simulink model "test_SimulinkMdl2_qLPVMPCbeta_UIO_inside"  (R2020a)
settings: Solver=FixedStepAuto  StartTime=0.0  StopTime=400  FixedStep=DT  RelTol=1e-3
values from neighbouring files (symbols this model uses):
  betaLUT = 0.0 0.064193209888351435 0.11259119004615419 0.14929546421559495 0.18081611050661253 0.20926497731412011 0.23701571242082992 0.26197392072434883 0.28536133270107289 0.30770154712660031 0.32934362985133 0.35028758087526196 0.37035886727319672 0.38973202197033374 0.40858157789187255    [DD_test.sldd]    (also in exUIO_WECS.m = unique(Lin_points.Pitch))
  DT = 0.008    [LUTMFile.m]    (also in UIOLinestTr.m; exUIO_WECS.m; getFictInputMatricesOrd3M.m; initWorkspace.m)
  lambdaCqVecLUT = 0.0 6.127061506348616E-5 0.00012254123012697232 0.00018381184519045848 0.00024508246025394464 0.00030635307531743077 0.00036762369038091696 0.00042889430544440315 0.00049016492050788928 0.00055143553557137541 0.00061270615063486154 0.00067397676569834778 0.00073524738076183392 0.00079651799582532 0.00085778861088880629 0.00091905922595229242 0.00098032984101577856 0.0010416004560792648 0.001102871    [DD_test.sldd]    (also in exUIO_WECS.m = lambdaCqVecMin : dLlambdaCqVec:lambdaCqVecMax)
  lambdaTildaMat = 14.419529569316524 14.349603210880673 12.133085869773012 9.9 8.4 7.3000000000000007 6.5 5.8000000000000007 5.4 4.9 4.6000000000000005 4.3 4.1000000000000005 3.9000000000000004 3.7 13.719392614649337 13.574357234178933 11.313379017594022 9.2598290519250313 7.9268106449449158 6.9824653636911407 6.2259000594299776 5.6530125740384722 5.1921371802911152 4.81807621242771 4.4910785109643978 4.22716815598    [DD_test.sldd]    (also in exUIO_WECS.m = lambdaCqVecMax *ones(size(lambdaCqMat)))
  Lin_points = 0.74811652133345019 0.78122947334555715 0.82586806925039735 0.88042797952230989 0.94564154658981237 1.06231329175348 1.1780905557148451 1.2402773842094346 1.254474305465946 1.2544764615597244 1.2544775037226534 1.2544778841663968 1.2544780221694662 1.2544779823335293 1.254477987181289 1.2544781738200332 1.254478189259095 1.2544780953600987 1.2544781548505395 1.2544783366942183 1.2544785605869417 1    [DD_test.sldd]    (also in LinPointsMFile.m = struct)
  sysEstTr : value not decoded    [DD_test.sldd]
  sysMeasDel : value not decoded    [DD_test.sldd]
  wecs = 3.0    [DD_test.sldd]    (also in MdlMFile.m = struct)
undefined symbols (not defined in the file or in its folder): Rotor_Lambda
libraries: sharedTrackingLibrary x1
settings Model: DataDictionary=DD_test.sldd  ExtModeTrigMode=oneshot  ExtModeArmWhenConnect=off  Creator=Hazim Namik  LastModifiedBy=ditt_aj
settings DataIOCC: LimitDataPoints=on  SaveFormat=Array  ReturnWorkspaceOutputs=off
settings OptimizationCC: BlockReduction=off  BooleanDataType=off  LifeSpan=inf
settings DebuggingCC: SaveWithParameterizedLinksMsg=none  UnderspecifiedInitializationDetection=Classic  MergeDetectMultiDrivingBlocksExec=none  SignalResolutionControl=TryResolveAllWithWarning  SFUnexpectedBacktrackingDiag=warning  SFNoUnconditionalDefaultTransitionDiag=warning  SFExecutionAtInitializationDiag=none  ArithmeticOperatorsInVariantConditions=warning
settings HardwareCC: ProdBitPerPointer=32  ProdBitPerSizeT=32  ProdBitPerPtrDiffT=32  ProdLargestAtomicFloat=None  ProdIntDivRoundTo=Undefined  ProdEndianess=Unspecified  ProdWordSize=32  ProdHWDeviceType=32-bit Generic  TargetUnknown=on
settings ModelReferenceCC: PropagateSignalLabelsOutOfModel=off
settings SFSimCC: SimUseLocalCustomCode=off  CustomCodeUndefinedFunction=UseInterfaceOnly
settings RTWCC: RTWUseLocalCustomCode=off
settings CodeAppCC: StateflowObjectComments=on
settings GRTTargetCC: TargetLangStandard=C89/C90 (ANSI)
settings ConfigComp: CovMetricSettings=dw  CovHtmlReporting=on  CovSaveCumulativeToWorkspaceVar=on  CovSaveSingleToWorkspaceVar=on  CovExternalEMLEnable=off

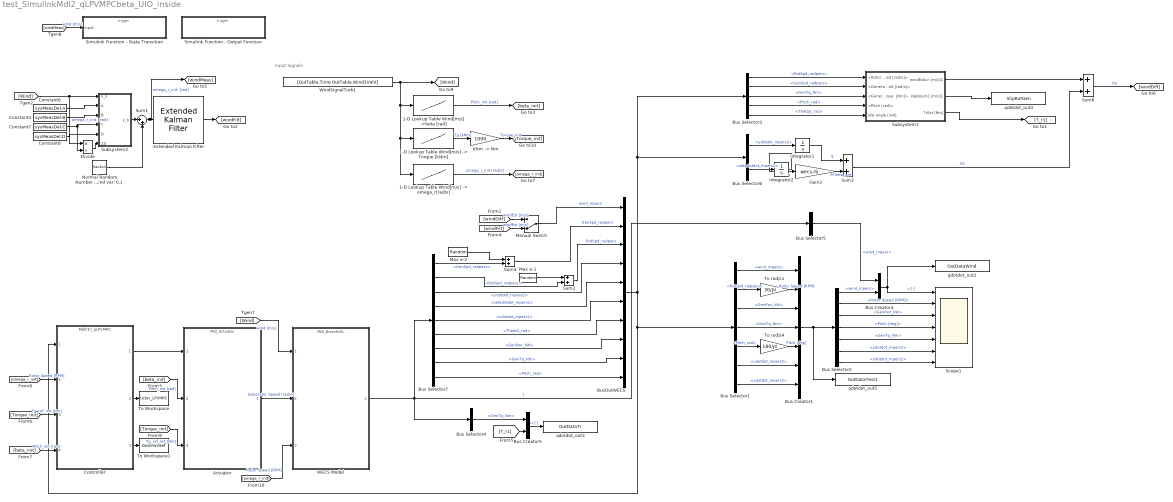
== system test_SimulinkMdl2_qLPVMPCbeta_UIO_inside ==
  note: Input Signals
  "1-D Lookup Table Wind[m/s] -> Torque [kNm]" : Lookup_n-D  NumberOfTableDimensions=1  BreakpointsForDimension1=Lin_points.V  BreakpointsForDimension2=Rotor_Lambda  Table=Lin_points.Torque  InternalRulePriority=Speed  RndMeth=Simplest  InputSameDT=on
  "1-D Lookup Table Wind[m/s] -> omega_r[rad/s]" : Lookup_n-D  NumberOfTableDimensions=1  BreakpointsForDimension1=Lin_points.V  BreakpointsForDimension2=Rotor_Lambda  Table=Lin_points.RSpeed  InternalRulePriority=Speed  RndMeth=Simplest  InputSameDT=on
  1-D Lookup Table Wind[m/s] ->beta [rad] : Lookup_n-D  NumberOfTableDimensions=1  BreakpointsForDimension1=Lin_points.V  BreakpointsForDimension2=Rotor_Lambda  Table=Lin_points.Pitch  InternalRulePriority=Speed  RndMeth=Simplest  InputSameDT=on
  Actuator : ModelReference  ModelNameDialog=Mdl_Actuator.slx  SimulationMode=Normal  ModelReferenceVersion=1.18
  Bus Creator1 : BusCreator  Inputs=7
  Bus Creator4 : BusCreator  Inputs=2
  Bus Creator5 : BusCreator  Inputs=2
  Bus Selector1 : BusSelector  OutputSignals=wind_mpers,RotSpd_radpers,GenPwr_kW,GenTq_Nm,Pitch_rad,ydotdot_mpers2,xdotdot_mpers2
  Bus Selector2 : BusSelector  OutputSignals=wind_mpers,Rotor Speed [RPM],GenPwr_kW,Pitch [deg],GenTq_Nm,ydotdot_mpers2,xdotdot_mpers2
  Bus Selector3 : BusSelector  OutputSignals=RotSpd_radpers,GenSpd_radpers,GenTq_Nm,Pitch_rad,ThetaS_rad
  Bus Selector4 : BusSelector  OutputSignals=GenTq_Nm
  Bus Selector5 : BusSelector  OutputSignals=wind_mpers
  Bus Selector6 : BusSelector  OutputSignals=ydotdot_mpers2,zetadotdot_mpers2
  Bus Selector7 : BusSelector  OutputSignals=GenSpd_radpers,RotSpd_radpers,ydotdot_mpers2,zetadotdot_mpers2,xdotdot_mpers2,ThetaS_rad,GenPwr_kW,GenTq_Nm,Pitch_rad
  BusOutWECS : BusCreator  Inputs=10  OutDataTypeStr=Bus: slBus1
  Constant4 : Constant  Value=sysMeasDel.B
  Constant6 : Constant  Value=sysMeasDel.A
  Constant7 : Constant  Value=sysMeasDel.C
  Constant8 : Constant  Value=sysMeasDel.D
  Controller : ModelReference  ModelNameDialog=MdlCtrl_qLPVMPC.slx  SimulationMode=Normal  ModelReferenceVersion=1.29
  Divide : Product  Inputs=*/
  Extended Kalman Filter : sharedTrackingLibrary/Extended Kalman Filter  StateTransitionFcn=stateTransitionFcn  HasStateTransitionJacobianFcn=off  StateTransitionJacobianFcn=stateTransitionJacobianFcn  HasAdditiveProcessNoise=Additive  ProcessNoise=0.1  HasTimeVaryingProcessNoise=off  HasStateTransitionFcnExtraArgument=0  InitialState=18  InitialStateCovariance=0.1  MeasurementFcn1=outputFcn  HasMeasurementJacobianFcn1=off  HasMeasurementEnablePort1=off  HasAdditiveMeasurementNoise1=Additive  MeasurementNoise1=1  HasTimeVaryingMeasurementNoise1=off  HasMeasurementFcnExtraArgument1=0  MeasurementFcn2=gpsMeasurementFcn  HasMeasurementJacobianFcn2=off  HasMeasurementEnablePort2=off  HasAdditiveMeasurementNoise2=Additive  MeasurementNoise2=[100 0; 0 100]  HasTimeVaryingMeasurementNoise2=off  HasMeasurementFcnExtraArgument2=0  MeasurementFcn3=myMeasurementFcn  HasMeasurementJacobianFcn3=off  HasMeasurementEnablePort3=off  HasAdditiveMeasurementNoise3=Additive  MeasurementNoise3=1  HasTimeVaryingMeasurementNoise3=off  HasMeasurementFcnExtraArgument3=0  MeasurementFcn4=myMeasurementFcn  HasMeasurementJacobianFcn4=off  HasMeasurementEnablePort4=off  HasAdditiveMeasurementNoise4=Additive  MeasurementNoise4=1  HasTimeVaryingMeasurementNoise4=off  HasMeasurementFcnExtraArgument4=0  MeasurementFcn5=myMeasurementFcn  HasMeasurementJacobianFcn5=off  HasMeasurementEnablePort5=off  HasAdditiveMeasurementNoise5=Additive  MeasurementNoise5=1  HasTimeVaryingMeasurementNoise5=off  HasMeasurementFcnExtraArgument5=0  EnableMultirate=off  StateTransitionFcnSampleTime=DT  MeasurementFcn1SampleTime=DT  MeasurementFcn2SampleTime=1  MeasurementFcn3SampleTime=-1  MeasurementFcn4SampleTime=-1  MeasurementFcn5SampleTime=-1  UseCurrentEstimator=off  OutputStateCovariance=off  DataType=double  SampleTime=DT  NumberOfMeasurements=1
      settings: SourceProductBaseCode=CT,DR,TF,ID,NV,AR,RO,VE
  Gain2 : Gain  Gain=wecs.rb
  Integrator1 : Integrator
  Integrator2 : Integrator
  Manual Switch : ManualSwitch  CurrentSetting=0
  Max e-1 : UniformRandomNumber  Minimum=-10^-4  Maximum=10^-4
  Max e-2 : UniformRandomNumber  Minimum=-10^-6  Maximum=10^-6
  Normal Random Number Wind var: 0.1 : RandomNumber  Variance=0.1  SampleTime=DT
  Scope1 : Scope  NumInputPorts=7
      settings: Tag=Scope
  Simulink Function - Output Function : Subsystem  TreatAsAtomicUnit=on
  Simulink Function - State Transition : Subsystem  TreatAsAtomicUnit=on
  Subsystem1 : Subsystem
  Subsystem2 : Subsystem
  Sum1 : Sum  Inputs=|++
  Sum{2..4,6} (4 alike) : Sum
  To Workspace : ToWorkspace  VariableName=tictoc_LPVMPC  SaveFormat=Timeseries  SampleTime=-1
  To Workspace1 : ToWorkspace  VariableName=GenPwrRef  SaveFormat=Timeseries  SampleTime=-1
  To rad/s1 : Gain  Gain=30/pi
  To rad/s4 : Gain  Gain=180/pi
  WECS Model : ModelReference  ModelNameDialog=Mdl_BianchiOL.slx  SimulationMode=Normal  ModelReferenceVersion=1.63
  WindSignalTurb1 : FromWorkspace  VariableName=[OutTable.Time OutTable.Wind1VelX]  SampleTime=DT  OutputAfterFinalValue=Holding final value
  "kNm -> Nm" : Gain  Gain=1000
  qdotdot_out2 : ToWorkspace  VariableName=OutDataWind  SampleTime=-1
  qdotdot_out3 : ToWorkspace  VariableName=OutDataTr  SampleTime=-1
  qdotdot_out4 : ToWorkspace  VariableName=SlipRotGen  SampleTime=-1
  qdotdot_out5 : ToWorkspace  VariableName=OutDataTest1  SampleTime=-1
  wires:
  WindSignalTurb1/1 -> [Wind], "1-D Lookup Table Wind[m/s] -> omega_r[rad/s]"/1, "1-D Lookup Table Wind[m/s] -> Torque [kNm]"/1, 1-D Lookup Table Wind[m/s] ->beta [rad]/1
  "kNm -> Nm"/1 -> [Torque_init]  "Torque_init"
  [omega_r_init] -> WECS Model/3  "Rotor Speed [RPM]"
  "1-D Lookup Table Wind[m/s] -> omega_r[rad/s]"/1 -> [omega_r_init]  "omega_r_init [rad/s]"
  [Wind] -> WECS Model/1  "wind [m/s]"
  1-D Lookup Table Wind[m/s] ->beta [rad]/1 -> [beta_init]  "Pitch_init [rad]"
  "1-D Lookup Table Wind[m/s] -> Torque [kNm]"/1 -> "kNm -> Nm"/1  "Tg [kNm]"
  Actuator/1 -> WECS Model/2  "Generator Speed [rad/s]"
  Controller/3 -> To Workspace1/1
  Bus Selector3/3 -> Subsystem1/3(<Generator Torque  [Nm]>)  "<GenTq_Nm>"
  Bus Selector3/4 -> Subsystem1/4(<Pitch [rad]>)  "<Pitch_rad>"
  Manual Switch/1 -> BusOutWECS/1  "wind_mpers"
  Bus Creator4/1 -> Scope1/1, qdotdot_out2/1  "u [-]"
  [Wind] -> Divide/1, Subsystem2/1(u_k)  "omega_r_init  [rad]"
  [windDiff] -> Manual Switch/1  "windEst [m/s]"
  Constant6/1 -> Subsystem2/2(A)
  Constant4/1 -> Subsystem2/3(B)
  Constant7/1 -> Subsystem2/4(C), Divide/2
  Constant8/1 -> Subsystem2/5(D)
  Divide/1 -> Subsystem2/6(Z0)
  Extended Kalman Filter/1 -> [windFilt]
  [windMeas] -> Simulink Function - State Transition/1(Input)  "wind [m/s]"
  Subsystem2/1(y_k) -> Sum1/1
  Sum1/1 -> [windMeas], Extended Kalman Filter/1  "omega_r_init  [rad]"
  Bus Selector3/5 -> Subsystem1/5(slip angle [rad])  "<ThetaS_rad>"
  Gain2/1 -> Sum3/2  "R*zeta_dot"
  Bus Selector6/1 -> Integrator1/1  "<ydotdot_mpers2>"
  Integrator1/1 -> Sum3/1  "q"
  Bus Selector6/2 -> Integrator2/1  "<zetadotdot_mpers2>"
  Integrator2/1 -> Gain2/1  "q"
  Sum3/1 -> Sum6/2  "Ve"
  Sum6/1 -> [windDiff]  "Ve"
  Subsystem1/1(windEstLin [m/s]1) -> Sum6/1
  Subsystem1/2(statesLIn2 [m/s]1) -> qdotdot_out4/1
  Subsystem1/3(TrEst [Nm]) -> [T_r1]
  Bus Creator5/1 -> qdotdot_out3/1  "u [-]"
  [T_r1] -> Bus Creator5/2
  Bus Selector3/2 -> Subsystem1/2(<Generator Speed [rad/s]>)  "<GenSpd_radpers>"
  Bus Selector3/1 -> Subsystem1/1(<Rotor Speed [rad/s]>)  "<RotSpd_radpers>"
  WECS Model/1 -> Bus Selector5/1, Bus Selector7/1, Bus Selector4/1  "]"
  [windFilt] -> Manual Switch/2  "windEst [m/s]"
  Normal Random Number Wind var: 0.1/1 -> Sum1/2
  Controller/2 -> To Workspace/1
  Controller/1 -> Actuator/1
  [beta_init] -> Actuator/2  "Pitch_init [rad]"
  [Torque_init] -> Actuator/3  "Tg_ref_init [Nm]"
  Bus Selector2/3 -> Scope1/3  "<GenPwr_kW>"
  Bus Selector2/7 -> Scope1/7  "<xdotdot_mpers2>"
  To rad/s4/1 -> Bus Creator1/5  "Pitch [deg]"
  Bus Selector2/4 -> Scope1/4  "<Pitch [deg]>"
  Bus Selector2/1 -> Bus Creator4/2  "<wind_mpers>"
  Bus Selector2/6 -> Scope1/6  "<ydotdot_mpers2>"
  Bus Selector1/5 -> To rad/s4/1  "<Pitch_rad>"
  Bus Selector1/4 -> Bus Creator1/4  "<GenTq_Nm>"
  Bus Selector2/2 -> Scope1/2  "<Rotor Speed [RPM]>"
  To rad/s1/1 -> Bus Creator1/2  "Rotor Speed [RPM]"
  Bus Selector1/6 -> Bus Creator1/6  "<ydotdot_mpers2>"
  Bus Selector2/5 -> Scope1/5  "<GenTq_Nm>"
  Bus Selector1/7 -> Bus Creator1/7  "<xdotdot_mpers2>"
  Bus Selector1/3 -> Bus Creator1/3  "<GenPwr_kW>"
  Max e-1/1 -> Sum2/1
  Bus Creator1/1 -> Bus Selector2/1, qdotdot_out5/1
  Max e-2/1 -> Sum4/1
  Bus Selector1/2 -> To rad/s1/1  "<RotSpd_radpers>"
  Bus Selector7/2 -> Sum2/2  "<RotSpd_radpers>"
  Bus Selector1/1 -> Bus Creator1/1  "<wind_mpers>"
  [Torque_init] -> Controller/3  "Tg_ref_init [Nm]"
  [beta_init] -> Controller/4  "Pitch_init [rad]"
  [omega_r_init] -> Controller/2  "Rotor Speed [RPM]"
  Bus Selector7/1 -> Sum4/2  "<GenSpd_radpers>"
  Sum4/1 -> BusOutWECS/2  "GenSpd_radpers"
  Sum2/1 -> BusOutWECS/3  "RotSpd_radpers"
  Bus Selector7/9 -> BusOutWECS/10  "<Pitch_rad>"
  Bus Selector7/8 -> BusOutWECS/9  "<GenTq_Nm>"
  Bus Selector7/7 -> BusOutWECS/8  "<GenPwr_kW>"
  Bus Selector7/6 -> BusOutWECS/7  "<ThetaS_rad>"
  Bus Selector7/5 -> BusOutWECS/6  "<xdotdot_mpers2>"
  Bus Selector7/4 -> BusOutWECS/5  "<zetadotdot_mpers2>"
  Bus Selector7/3 -> BusOutWECS/4  "<ydotdot_mpers2>"
  Bus Selector4/1 -> Bus Creator5/1  "<GenTq_Nm>"
  BusOutWECS/1 -> Bus Selector6/1, Bus Selector3/1, Bus Selector1/1, Controller/1
  Bus Selector5/1 -> Bus Creator4/1  "<wind_mpers>"

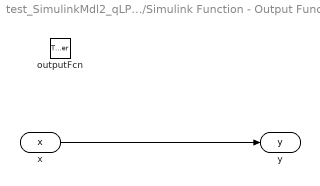
== system test_SimulinkMdl2_qLPVMPCbeta_UIO_inside/Simulink Function - Output Function ==
  outputFcn : TriggerPort  TriggerType=function-call  IsSimulinkFunction=on  FunctionName=outputFcn  VariantControl=Variant
  x : ArgIn  DisableCoverage=on  ArgumentName=x
  y : ArgOut  DisableCoverage=on  ArgumentName=y
  wires:
  x/1 -> y/1

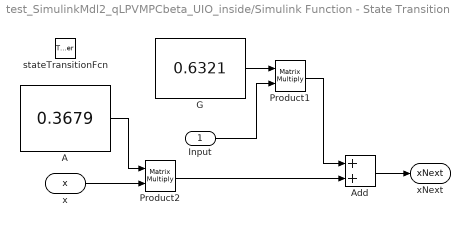
== system test_SimulinkMdl2_qLPVMPCbeta_UIO_inside/Simulink Function - State Transition ==
  Input : Inport
  stateTransitionFcn : TriggerPort  TriggerType=function-call  IsSimulinkFunction=on  FunctionName=stateTransitionFcn  VariantControl=Variant
  A : Constant  Value=0.3679
  Add : Sum
  G : Constant  Value=0.6321
  Product1 : Product  Multiplication=Matrix(*)
  Product2 : Product  Multiplication=Matrix(*)
  x : ArgIn  DisableCoverage=on  ArgumentName=x
  xNext : ArgOut  DisableCoverage=on  ArgumentName=xNext
  wires:
  x/1 -> Product2/2
  A/1 -> Product2/1
  Product2/1 -> Add/2
  G/1 -> Product1/1
  Input/1 -> Product1/2
  Product1/1 -> Add/1
  Add/1 -> xNext/1

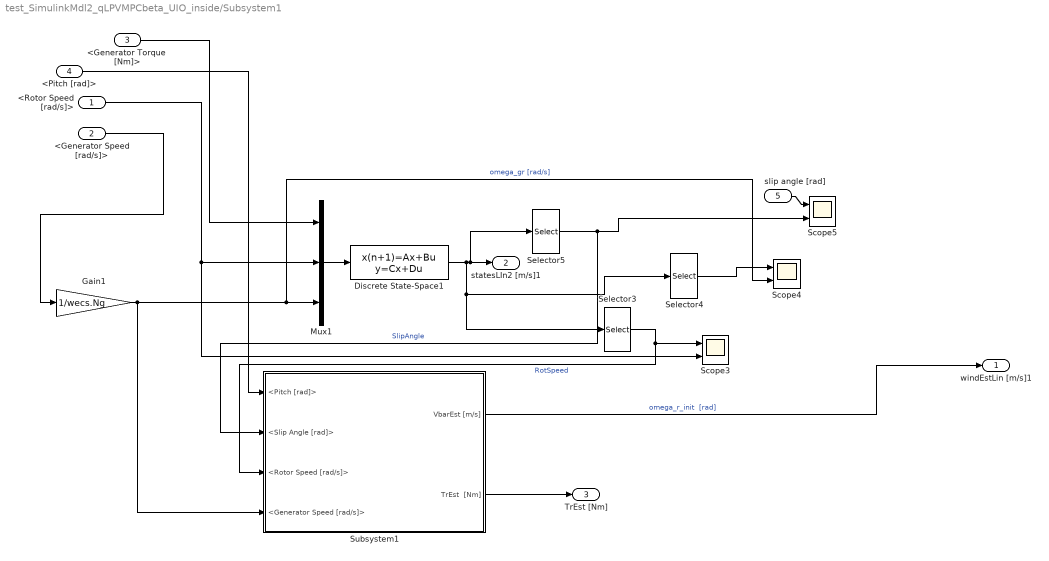
== system test_SimulinkMdl2_qLPVMPCbeta_UIO_inside/Subsystem1 ==
  <Rotor Speed [rad/s]> : Inport
  <Generator Speed [rad/s]> : Inport  Port=2
  <Generator Torque  [Nm]> : Inport  Port=3
  <Pitch [rad]> : Inport  Port=4
  slip angle [rad] : Inport  Port=5
  Discrete State-Space1 : DiscreteStateSpace  A=sysEstTr.A  B=sysEstTr.B  C=sysEstTr.C  D=sysEstTr.D  InitialCondition=[0,0,1.25]  SampleTime=DT
  Gain1 : Gain  Gain=1/wecs.Ng
  Mux1 : Mux  Inputs=3
  Scope3 : Scope  NumInputPorts=2
  Scope4 : Scope  NumInputPorts=2
  Scope5 : Scope  NumInputPorts=2
  Selector3 : Selector  InputPortWidth=3  IndexOptions=Index vector (dialog)  Indices=2  OutputSizes=1
  Selector4 : Selector  InputPortWidth=3  IndexOptions=Index vector (dialog)  Indices=3  OutputSizes=1
  Selector5 : Selector  InputPortWidth=3  IndexOptions=Index vector (dialog)  Indices=1  OutputSizes=1
  Subsystem1 : Subsystem
  windEstLin [m/s]1 : Outport
  statesLIn2 [m/s]1 : Outport  Port=2
  TrEst [Nm] : Outport  Port=3
  wires:
  <Generator Speed [rad/s]>/1 -> Gain1/1
  <Generator Torque  [Nm]>/1 -> Mux1/1
  <Pitch [rad]>/1 -> Subsystem1/1(<Pitch [rad]>)
  slip angle [rad]/1 -> Scope5/1
  Subsystem1/1(VbarEst [m/s]) -> windEstLin [m/s]1/1  "omega_r_init  [rad]"
  <Rotor Speed [rad/s]>/1 -> Mux1/2, Scope3/2
  Mux1/1 -> Discrete State-Space1/1
  Selector3/1 -> Subsystem1/3(<Rotor Speed [rad/s]>), Scope3/1  "RotSpeed"
  Gain1/1 -> Subsystem1/4(<Generator Speed [rad/s]>), Scope4/2, Mux1/3  "omega_gr [rad/s]"
  Discrete State-Space1/1 -> Selector5/1, statesLIn2 [m/s]1/1, Selector4/1, Selector3/1
  Selector4/1 -> Scope4/1
  Selector5/1 -> Subsystem1/2(<Slip Angle [rad]>), Scope5/2  "SlipAngle"
  Subsystem1/2(TrEst  [Nm]) -> TrEst [Nm]/1

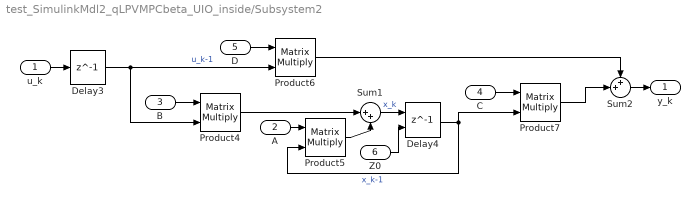
== system test_SimulinkMdl2_qLPVMPCbeta_UIO_inside/Subsystem2 ==
  u_k : Inport
  A : Inport  Port=2
  B : Inport  Port=3
  C : Inport  Port=4
  D : Inport  Port=5
  Z0 : Inport  Port=6
  Delay3 : Delay  DelayLength=1
  Delay4 : Delay  DelayLength=1  InitialConditionSource=Input port
      settings: InputPortMap=u0,p4
  Product{4..7} (4 alike) : Product  Multiplication=Matrix(*)
  Sum1 : Sum  Inputs=|++
  Sum2 : Sum  Inputs=++|
  y_k : Outport
  wires:
  Delay4/1 -> Product7/2, Product5/2  "x_k-1"
  u_k/1 -> Delay3/1
  Product7/1 -> Sum2/2
  C/1 -> Product7/1
  Product6/1 -> Sum2/1
  Delay3/1 -> Product4/2, Product6/2  "u_k-1"
  Product5/1 -> Sum1/2
  D/1 -> Product6/1
  Product4/1 -> Sum1/1
  A/1 -> Product5/1
  Sum1/1 -> Delay4/1  "x_k"
  B/1 -> Product4/1
  Sum2/1 -> y_k/1
  Z0/1 -> Delay4/2

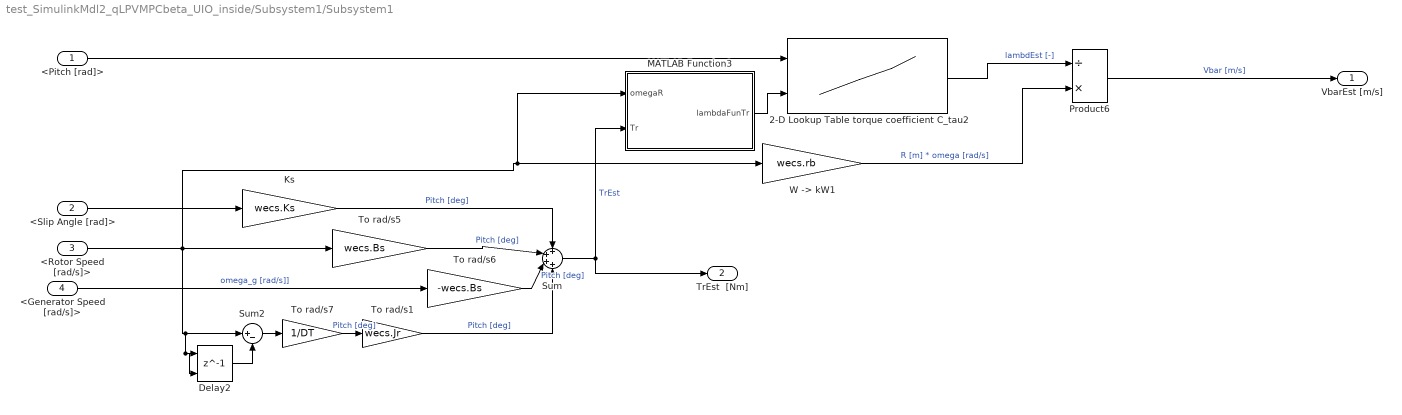
== system test_SimulinkMdl2_qLPVMPCbeta_UIO_inside/Subsystem1/Subsystem1 ==
  <Pitch [rad]> : Inport
  <Slip Angle [rad]> : Inport  Port=2
  <Rotor Speed [rad/s]> : Inport  Port=3
  <Generator Speed [rad/s]> : Inport  Port=4
  2-D Lookup Table torque coefficient C_tau2 : Lookup_n-D  BreakpointsForDimension1=betaLUT  BreakpointsForDimension2=lambdaCqVecLUT  Table=lambdaTildaMat  InterpMethod=Cubic spline  InternalRulePriority=Speed  RndMeth=Simplest  InputSameDT=on
  Delay2 : Delay  DelayLength=1  InitialConditionSource=Input port  InitialCondition=0
      settings: InputPortMap=u0,p4
  Ks : Gain  Gain=wecs.Ks
  MATLAB Function3 : MATLAB Function  TreatAsAtomicUnit=on
  Product6 : Product  Inputs=/*
  Sum : Sum  Inputs=4
  Sum2 : Sum  Inputs=|+-
  To rad/s1 : Gain  Gain=wecs.Jr
  To rad/s5 : Gain  Gain=wecs.Bs
  To rad/s6 : Gain  Gain=-wecs.Bs
  To rad/s7 : Gain  Gain=1/DT
  "W -> kW1" : Gain  Gain=wecs.rb
  VbarEst [m/s] : Outport
  TrEst  [Nm] : Outport  Port=2
  wires:
  2-D Lookup Table torque coefficient C_tau2/1 -> Product6/1  "lambdEst [-]"
  To rad/s1/1 -> Sum/4  "Pitch [deg]"
  Product6/1 -> VbarEst [m/s]/1  "Vbar [m/s]"
  Sum/1 -> MATLAB Function3/2(Tr), TrEst  [Nm]/1  "TrEst"
  <Rotor Speed [rad/s]>/1 -> To rad/s5/1, "W -> kW1"/1, MATLAB Function3/1(omegaR), Delay2/1, Delay2/2, Sum2/1
  Sum2/1 -> To rad/s7/1
  To rad/s5/1 -> Sum/2  "Pitch [deg]"
  Delay2/1 -> Sum2/2
  MATLAB Function3/1(lambdaFunTr) -> 2-D Lookup Table torque coefficient C_tau2/2
  <Generator Speed [rad/s]>/1 -> To rad/s6/1  "omega_g [rad/s]]"
  To rad/s7/1 -> To rad/s1/1  "Pitch [deg]"
  To rad/s6/1 -> Sum/3  "Pitch [deg]"
  <Pitch [rad]>/1 -> 2-D Lookup Table torque coefficient C_tau2/1
  Ks/1 -> Sum/1  "Pitch [deg]"
  "W -> kW1"/1 -> Product6/2  "R [m] * omega [rad/s]"
  <Slip Angle [rad]>/1 -> Ks/1

== matlab function test_SimulinkMdl2_qLPVMPCbeta_UIO_inside/Subsystem1/Subsystem1/MATLAB Function3 ==
  data: omegaR input; Tr input; lambdaFunTr output
function lambdaFunTr = getlambdaFunTr(omegaR,Tr)

rho = 1.2250; % air density
rb = 63; % m blade radius

lambdaFunTr = 2* Tr /(rho *pi * rb^5*omegaR^2);
